simulink model "YMBOX_Control_Core"  (R2024b)
settings: Solver=FixedStepDiscrete  StartTime=0.0  StopTime=3  RelTol=1e-3
PreLoadFcn:
  | run(fullfile(fileparts(get_param(bdroot,'FileName')), 'YMBOX_Deluxe_init.m'));
InitFcn:
  | YMBOX_InitializeModel('core',bdroot);
model workspace (MAT data in the model file):
  KuMDAS_ObserverBuildVariant : Simulink.Parameter (value not decoded)
undefined symbols (not defined in the file or in its folder): CeMDSM_DrvModeIfStart_enum, CeMDSM_DrvModeSpdSens_enum, CeMDSM_DrvModeSpdSmo_enum, CeMDSM_DrvModeTrq_enum, Cf_CONTROL_TASK_TIME_S, KbMDAS_SmoDeadTimeCompEnable_flg, KbMDSA_ActiveInverterCompEnable_flg, KbMDSA_UnifiedVoltageLimitEnable_flg, KbMDSP_DCBusVoltReportFilterEnable_flg, KbMDTM_DAxisPriorityInFW_flg, KbMDTM_FieldWeakeningEnable_flg, KbMDTM_FinalIqAntiWindupEnable_flg, KbMDTM_SensorlessFieldWeakeningEnable_flg, KbMDTM_TorquePriorityBelowBase_flg, KbMDTM_UnifiedConstraintEnable_flg, KfMDAS_ControlCountToElecRad_NULL, KfMDAS_IfAccel_rpms, KfMDAS_IfAlignTime_s, KfMDAS_IfBlendTime_s, KfMDAS_IfSwitchSpd_rpm, KfMDAS_NativeCountToMechRad_NULL, KfMDAS_ObserverExitRatio_NULL, KfMDAS_SlsCtrlPeriod_s, KfMDAS_SlsEAngleInit_rad, KfMDAS_SlsElecSpdMax_rads, KfMDAS_SlsElecSpdMin_rads, KfMDAS_SlsTwoPi_rad, KfMDAS_SmoAngleOffset_rad, KfMDAS_SmoCurrentZohCoefA_NULL, KfMDAS_SmoCurrentZohCoefB_AperV, KfMDAS_SmoDeadTimeCurrentBoundary_A, KfMDAS_SmoDeadTimeDuty_NULL, KfMDAS_SmoDeadTimePolarity_NULL, KfMDAS_SmoDeviceDrop_V, KfMDAS_SmoEmfLpfCoefA_NULL, KfMDAS_SmoEmfLpfCoefB_NULL, KfMDAS_SmoEmfLpfInvPole_s, KfMDAS_SmoErrBoundaryMax_A, KfMDAS_SmoErrBoundarySpan_A, KfMDAS_SmoGainSchedAlpha_NULL, KfMDAS_SmoGainSchedAngleComp_rad, KfMDAS_SmoGainSchedEmfLow_V, KfMDAS_SmoGainSchedInvSpan_PerV, KfMDAS_SmoLdMinusLq_H, KfMDAS_SmoPllKiTs_NULL, KfMDAS_SmoPllKp_NULL, KfMDAS_SmoPllMinEmf_V, KfMDAS_SmoPllSpeedLpfAlpha_NULL, KfMDAS_SmoSlideGainMin_V, KfMDAS_SmoSlideGainSpan_V, KfMDAS_SmoSwitchSpd_rpm, KfMDAS_SmoTotalDelay_s, KfMDCC_DqSoftwareOverCurrentThreshold_A, KfMDCC_PiKcTsId_NULL, KfMDCC_PiKcTsIq_NULL, KfMDCC_PiKiTsId_NULL, KfMDCC_PiKiTsIq_NULL, KfMDCC_PiKpValueId_NULL, KfMDCC_PiKpValueIq_NULL, KfMDCC_PwmFreq_Hz ... (+84)
libraries: YMBOX_SharedMath_Lib x11, spsabctoAlphaBetaZeroLib x1
(part 3 of 8)

== system YMBOX_Control_Core/MDSP/Phase_Current_Conditioning ==
  phaseU_A : Inport  OutDataTypeStr=single
  phaseV_A : Inport  Port=2  OutDataTypeStr=single
  phaseW_A : Inport  Port=3  OutDataTypeStr=single
  phaseUError_flg : Inport  Port=4  OutDataTypeStr=boolean
  phaseVError_flg : Inport  Port=5  OutDataTypeStr=boolean
  phaseWError_flg : Inport  Port=6  OutDataTypeStr=boolean
  Invalid : Logic  Operator=OR  Inputs=3  IconShape=distinctive
  Pair0 : Logic  IconShape=distinctive
  Pair1 : Logic  IconShape=distinctive
  Pair2 : Logic  IconShape=distinctive
  Reconstruct0 : Sum  Inputs=--
  Reconstruct1 : Sum  Inputs=--
  Reconstruct2 : Sum  Inputs=--
  Safe0 : Switch  Criteria=u2 ~= 0
  Safe1 : Switch  Criteria=u2 ~= 0
  Safe2 : Switch  Criteria=u2 ~= 0
  Single0 : Switch  Criteria=u2 ~= 0
  Single1 : Switch  Criteria=u2 ~= 0
  Single2 : Switch  Criteria=u2 ~= 0
  Zero : Constant  Value=single(0)  OutDataTypeStr=single
  VfMDSP_PhaseUCurrentCtrl_A : Outport
  VfMDSP_PhaseVCurrentCtrl_A : Outport  Port=2
  VfMDSP_PhaseWCurrentCtrl_A : Outport  Port=3
  wires:
  phaseUError_flg/1 -> Single0/2, Pair0/1, Pair1/1
  Reconstruct0/1 -> Single0/1
  phaseU_A/1 -> Reconstruct2/1, Single0/3, Reconstruct1/1
  phaseVError_flg/1 -> Pair0/2, Pair2/1, Single1/2
  phaseWError_flg/1 -> Pair1/2, Pair2/2, Single2/2
  phaseV_A/1 -> Reconstruct2/2, Single1/3, Reconstruct0/1
  Pair0/1 -> Invalid/1
  phaseW_A/1 -> Single2/3, Reconstruct0/2, Reconstruct1/2
  Pair1/1 -> Invalid/2
  Pair2/1 -> Invalid/3
  Reconstruct2/1 -> Single2/1
  Reconstruct1/1 -> Single1/1
  Single0/1 -> Safe0/3
  Zero/1 -> Safe0/1, Safe2/1, Safe1/1
  Invalid/1 -> Safe0/2, Safe2/2, Safe1/2
  Single2/1 -> Safe2/3
  Single1/1 -> Safe1/3
  Safe0/1 -> VfMDSP_PhaseUCurrentCtrl_A/1
  Safe2/1 -> VfMDSP_PhaseWCurrentCtrl_A/1
  Safe1/1 -> VfMDSP_PhaseVCurrentCtrl_A/1

== system YMBOX_Control_Core/MDSP/Resolver_Processing ==
  VuMINP_ResolverPositionRaw_NULL : Inport  OutDataTypeStr=uint32
  ControlAngleCounts : Constant  Value=KfPLL_ControlAngleCounts_NULL
  ElectricAngle_ToUint16 : DataTypeConversion  OutDataTypeStr=uint16
  MechanicalRaw_Uint32 : SignalConversion  OverrideOpt=off
  NativeToElectricalCounts : Gain  Gain=KfPLL_PolePairsNativeToControl_NULL  OutDataTypeStr=single  SaturateOnIntegerOverflow=on
  Resolver_Output_Bus : BusCreator  Inputs=2  OutDataTypeStr=Bus: Resolver_Output  NonVirtualBus=on
      settings: InheritFromInputs=off
  WrapElectricalCount : Math  Operator=mod  OutDataTypeStr=uint16
  Resolver_Output : Outport  OutDataTypeStr=Bus: Resolver_Output
  wires:
  Resolver_Output_Bus/1 -> Resolver_Output/1  "Resolver_Output"
  MechanicalRaw_Uint32/1 -> Resolver_Output_Bus/2  "VuMDSP_MotMechAngleRaw_NULL"
  ElectricAngle_ToUint16/1 -> Resolver_Output_Bus/1  "VuMDSP_MotEAngle_NULL"
  VuMINP_ResolverPositionRaw_NULL/1 -> NativeToElectricalCounts/1, MechanicalRaw_Uint32/1
  NativeToElectricalCounts/1 -> WrapElectricalCount/1
  ControlAngleCounts/1 -> WrapElectricalCount/2
  WrapElectricalCount/1 -> ElectricAngle_ToUint16/1

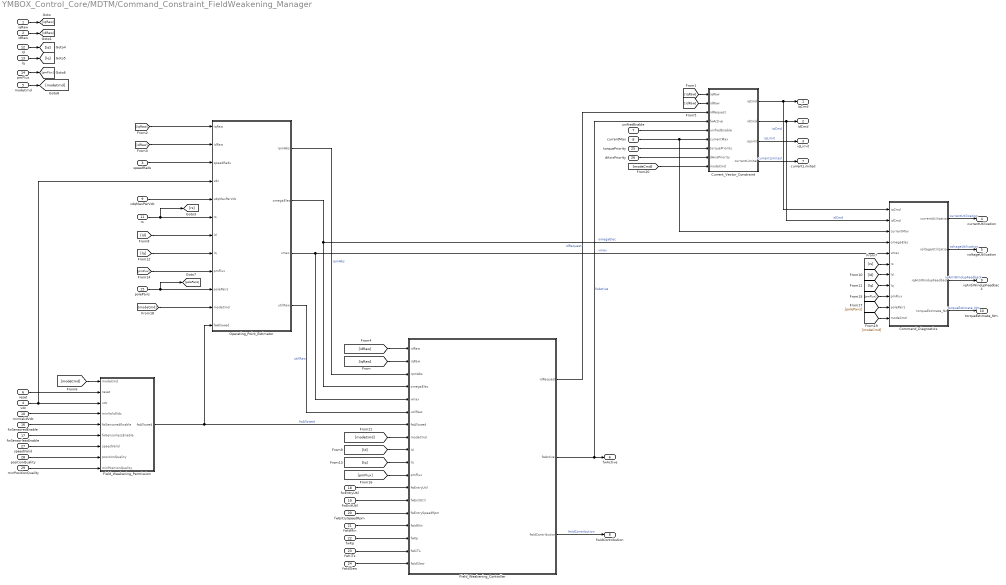
== system YMBOX_Control_Core/MDTM/Command_Constraint_FieldWeakening_Manager ==
  iqRaw : Inport
  idRaw : Inport  Port=2
  speedRads : Inport  Port=3
  vdc : Inport  Port=4
  modeCmd : Inport  Port=5
  reset : Inport  Port=6
  unifiedEnable : Inport  Port=7
  currentMax : Inport  Port=8
  vdqMaxPerVdc : Inport  Port=9
  minValidVdc : Inport  Port=10
  rs : Inport  Port=11
  ld : Inport  Port=12
  lq : Inport  Port=13
  pmFlux : Inport  Port=14
  polePairs : Inport  Port=15
  fwSensoredEnable : Inport  Port=16
  fwSensorlessEnable : Inport  Port=17
  fwEntryUtil : Inport  Port=18
  fwExitUtil : Inport  Port=19
  fwEntrySpeedRpm : Inport  Port=20
  fwIdMin : Inport  Port=21
  fwKp : Inport  Port=22
  fwKiTs : Inport  Port=23
  fwIdSlew : Inport  Port=24
  torquePriority : Inport  Port=25
  dAxisPriority : Inport  Port=26
  speedValid : Inport  Port=27
  positionQuality : Inport  Port=28
  minPositionQuality : Inport  Port=29
  Command_Diagnostics : Subsystem
  Current_Vector_Constraint : Subsystem
  Field_Weakening_Controller : Subsystem
  Field_Weakening_Permission : Subsystem
  Operating_Point_Estimator : Subsystem
  iqCmd : Outport
  idCmd : Outport  Port=2
  iqLimit : Outport  Port=3
  currentUtilization : Outport  Port=4
  voltageUtilization : Outport  Port=5
  fwActive : Outport  Port=6
  currentLimited : Outport  Port=7
  fwIdContribution : Outport  Port=8
  iqAntiWindupFeedback : Outport  Port=9
  torqueEstimate_Nm : Outport  Port=10
  wires:
  vdqMaxPerVdc/1 -> Operating_Point_Estimator/5(vdqMaxPerVdc)
  reset/1 -> Field_Weakening_Permission/2(reset)
  Operating_Point_Estimator/2(omegaElec) -> Field_Weakening_Controller/4(omegaElec), Command_Diagnostics/4(omegaElec)  "omegaElec"
  Command_Diagnostics/2(voltageUtilization) -> voltageUtilization/1  "voltageUtilization"
  vdc/1 -> Operating_Point_Estimator/4(vdc), Field_Weakening_Permission/3(vdc)
  speedRads/1 -> Operating_Point_Estimator/3(speedRads)
  Command_Diagnostics/4(torqueEstimate_Nm) -> torqueEstimate_Nm/1  "torqueEstimate_Nm"
  Operating_Point_Estimator/4(utilRaw) -> Field_Weakening_Controller/6(utilRaw)  "utilRaw"
  rs/1 -> [rs], Operating_Point_Estimator/6(rs)
  Current_Vector_Constraint/4(currentLimited) -> currentLimited/1  "currentLimited"
  Field_Weakening_Controller/2(fwActive) -> fwActive/1, Current_Vector_Constraint/4(fwActive)  "fwActive"
  polePairs/1 -> [polePairs], Operating_Point_Estimator/10(polePairs)
  Operating_Point_Estimator/1(rpmAbs) -> Field_Weakening_Controller/3(rpmAbs)  "rpmAbs"
  Operating_Point_Estimator/3(vmax) -> Field_Weakening_Controller/5(vmax), Command_Diagnostics/5(vmax)  "vmax"
  fwEntryUtil/1 -> Field_Weakening_Controller/12(fwEntryUtil)
  Current_Vector_Constraint/2(idCmd) -> Command_Diagnostics/2(idCmd), idCmd/1  "idCmd"
  fwExitUtil/1 -> Field_Weakening_Controller/13(fwExitUtil)
  fwEntrySpeedRpm/1 -> Field_Weakening_Controller/14(fwEntrySpeedRpm)
  fwIdMin/1 -> Field_Weakening_Controller/15(fwIdMin)
  fwKp/1 -> Field_Weakening_Controller/16(fwKp)
  fwKiTs/1 -> Field_Weakening_Controller/17(fwKiTs)
  fwIdSlew/1 -> Field_Weakening_Controller/18(fwIdSlew)
  unifiedEnable/1 -> Current_Vector_Constraint/5(unifiedEnable)
  torquePriority/1 -> Current_Vector_Constraint/7(torquePriority)
  dAxisPriority/1 -> Current_Vector_Constraint/8(dAxisPriority)
  currentMax/1 -> Command_Diagnostics/3(currentMax), Current_Vector_Constraint/6(currentMax)
  Field_Weakening_Controller/1(idRequest) -> Current_Vector_Constraint/3(idRequest)  "idRequest"
  Command_Diagnostics/1(currentUtilization) -> currentUtilization/1  "currentUtilization"
  Field_Weakening_Controller/3(fwIdContribution) -> fwIdContribution/1  "fwIdContribution"
  Current_Vector_Constraint/1(iqCmd) -> Command_Diagnostics/1(iqCmd), iqCmd/1  "iqCmd"
  Current_Vector_Constraint/3(iqLimit) -> iqLimit/1  "iqLimit"
  Command_Diagnostics/3(iqAntiWindupFeedback) -> iqAntiWindupFeedback/1  "iqAntiWindupFeedback"
  iqRaw/1 -> [iqRaw]
  [iqRaw] -> Field_Weakening_Controller/2(iqRaw)
  [iqRaw] -> Current_Vector_Constraint/1(iqRaw)
  [iqRaw] -> Operating_Point_Estimator/1(iqRaw)
  idRaw/1 -> [idRaw]
  [idRaw] -> Operating_Point_Estimator/2(idRaw)
  [idRaw] -> Field_Weakening_Controller/1(idRaw)
  [idRaw] -> Current_Vector_Constraint/2(idRaw)
  [rs] -> Command_Diagnostics/6(rs)
  ld/1 -> [ld]
  [ld] -> Operating_Point_Estimator/7(ld)
  [ld] -> Field_Weakening_Controller/9(ld)
  [ld] -> Command_Diagnostics/7(ld)
  lq/1 -> [lq]
  [lq] -> Command_Diagnostics/8(lq)
  [lq] -> Operating_Point_Estimator/8(lq)
  [lq] -> Field_Weakening_Controller/10(lq)
  pmFlux/1 -> [pmFlux]
  [pmFlux] -> Operating_Point_Estimator/9(pmFlux)
  [pmFlux] -> Command_Diagnostics/9(pmFlux)
  [pmFlux] -> Field_Weakening_Controller/11(pmFlux)
  [polePairs] -> Command_Diagnostics/10(polePairs)
  modeCmd/1 -> [modeCmd]
  [modeCmd] -> Operating_Point_Estimator/11(modeCmd)
  [modeCmd] -> Command_Diagnostics/11(modeCmd)
  [modeCmd] -> Current_Vector_Constraint/9(modeCmd)
  [modeCmd] -> Field_Weakening_Controller/8(modeCmd)
  minValidVdc/1 -> Field_Weakening_Permission/4(minValidVdc)
  fwSensoredEnable/1 -> Field_Weakening_Permission/5(fwSensoredEnable)
  fwSensorlessEnable/1 -> Field_Weakening_Permission/6(fwSensorlessEnable)
  speedValid/1 -> Field_Weakening_Permission/7(speedValid)
  positionQuality/1 -> Field_Weakening_Permission/8(positionQuality)
  minPositionQuality/1 -> Field_Weakening_Permission/9(minPositionQuality)
  Field_Weakening_Permission/1(fwAllowed) -> Operating_Point_Estimator/12(fwAllowed), Field_Weakening_Controller/7(fwAllowed)  "fwAllowed"
  [modeCmd] -> Field_Weakening_Permission/1(modeCmd)

== system YMBOX_Control_Core/MDTM/MDTM ==
  note: 1) Add Subsystem or Model blocks as valid variant choices.
      | 2) You cannot connect blocks at this level. At simulation, connectivity is automatically
      | determined, based on the active variant and port name matching.
  VeMDTM_DrvModeCmd_enum : Inport
  VeMDTM_DrvModeReq_enum : Inport  Port=2
  VfMDTM_SpdCmd_rpm : Inport  Port=3
  VfMDTM_TrqCmd_Nm : Inport  Port=4
  VbMDCC_PiReset_flg : Inport  Port=5
  VfMDCC_TestUalphaUdId_NULL : Inport  Port=6
  VfMDTM_TestUbetaUqIq_NULL : Inport  Port=7
  VfMDTM_HandoverBlend_NULL : Inport  Port=8
  VfMDTM_HandoverElecAngleDelta_rad : Inport  Port=9
  VfMDTM_MotMechSpdFiltered_rads : Inport  Port=10
  VfMDTM_MotElecAngle_rad : Inport  Port=11
  VfMDTM_PhaseUCur_A : Inport  Port=12
  VfMDTM_PhaseVCur_A : Inport  Port=13
  VfMDTM_PhaseWCur_A : Inport  Port=14
  VfMDTM_ExecutionScale_NULL : Inport  Port=15  OutDataTypeStr=single
  MDTM_SMO : Subsystem  TreatAsAtomicUnit=on  VariantControl=KuMDAS_ObserverBuildVariant == 1
      settings: AttributesFormatString=PRODUCT TORQUE/SPEED CONTROL\nMODE 6: SENSORLESS SPEED
  MDTM_SensoredOnly : Subsystem  TreatAsAtomicUnit=on  VariantControl=KuMDAS_ObserverBuildVariant == 0
      settings: AttributesFormatString=|
      | SENSORED ONLY
      | Original direct voltage/speed/torque modes 3/4/5
  MDTM_outputs : Outport

== system YMBOX_Control_Core/MDTM/MotorCurrentReferenceGenerator ==
  note: 1) Add Subsystem or Model blocks as valid variant choices.
      | 2) You cannot connect blocks at this level. At simulation, connectivity is automatically
      | determined, based on the active variant and port name matching.
  modeCmd_enum : Inport
  iqLegacy_A : Inport  Port=2
  idLegacy_A : Inport  Port=3
  handoverBlend_NULL : Inport  Port=4  OutDataTypeStr=single
  MotorCurrentReference_IPMSM : Subsystem  VariantControl=KuMDTM_MotorCurrentReferenceVariant == 1
  MotorCurrentReference_SPMSM : Subsystem  VariantControl=KuMDTM_MotorCurrentReferenceVariant == 0
  iqReference_A : Outport
  idReference_A : Outport  Port=2
  torqueRequest_Nm : Outport  Port=3
  mtpaActive_flg : Outport  Port=4

== system YMBOX_Control_Core/MDAS/IF_Startup_Internal/IF_Startup_SMO ==
  VeMDAS_DrvModeCmd_enum : Inport
  VeMDAS_DrvModeReq_enum : Inport  Port=2
  VfMDAS_TargetSpd_rpm : Inport  Port=3
  VfMDAS_SmoElecSpd_rads : Inport  Port=4
  VfMDAS_SmoElecAngle_rad : Inport  Port=5
  VfMDAS_SmoEmfMag_V : Inport  Port=6
  VfMDAS_SmoPllPhaseErr_NULL : Inport  Port=7
  SMO_ProductMode_Core : Stateflow chart  TreatAsAtomicUnit=on
  VfMDAS_IfMechSpd_rads : Outport
  VfMDAS_IfMechSpdAbs_rads : Outport  Port=2
  VfMDAS_IfElecAngle_rad : Outport  Port=3
  VfMDAS_SmoMechSpd_rads : Outport  Port=4
  VfMDAS_SmoMechSpdAbs_rads : Outport  Port=5
  VbMDAS_SmoReady_flg : Outport  Port=6
  VfMDAS_SmoAlignedElecAngle_rad : Outport  Port=7
  VfMDAS_HandoverBlend_NULL : Outport  Port=8
  VfMDAS_HandoverElecAngleDelta_rad : Outport  Port=9
  wires:
  VeMDAS_DrvModeCmd_enum/1 -> SMO_ProductMode_Core/1(VeMDAS_DrvModeCmd_enum)
  VeMDAS_DrvModeReq_enum/1 -> SMO_ProductMode_Core/2(VeMDAS_DrvModeReq_enum)
  SMO_ProductMode_Core/2(VfMDAS_IfMechSpdAbs_rads) -> VfMDAS_IfMechSpdAbs_rads/1
  SMO_ProductMode_Core/1(VfMDAS_IfMechSpd_rads) -> VfMDAS_IfMechSpd_rads/1
  VfMDAS_TargetSpd_rpm/1 -> SMO_ProductMode_Core/3(VfMDAS_TargetSpd_rpm)
  VfMDAS_SmoElecSpd_rads/1 -> SMO_ProductMode_Core/4(VfMDAS_SmoElecSpd_rads)
  VfMDAS_SmoElecAngle_rad/1 -> SMO_ProductMode_Core/5(VfMDAS_SmoElecAngle_rad)
  VfMDAS_SmoEmfMag_V/1 -> SMO_ProductMode_Core/6(VfMDAS_SmoEmfMag_V)
  VfMDAS_SmoPllPhaseErr_NULL/1 -> SMO_ProductMode_Core/7(VfMDAS_SmoPllPhaseErr_NULL)
  SMO_ProductMode_Core/6(VbMDAS_SmoReady_flg) -> VbMDAS_SmoReady_flg/1
  SMO_ProductMode_Core/5(VfMDAS_SmoMechSpdAbs_rads) -> VfMDAS_SmoMechSpdAbs_rads/1
  SMO_ProductMode_Core/4(VfMDAS_SmoMechSpd_rads) -> VfMDAS_SmoMechSpd_rads/1
  SMO_ProductMode_Core/3(VfMDAS_IfElecAngle_rad) -> VfMDAS_IfElecAngle_rad/1
  SMO_ProductMode_Core/9(VfMDAS_HandoverElecAngleDelta_rad) -> VfMDAS_HandoverElecAngleDelta_rad/1
  SMO_ProductMode_Core/8(VfMDAS_HandoverBlend_NULL) -> VfMDAS_HandoverBlend_NULL/1
  SMO_ProductMode_Core/7(VfMDAS_SmoAlignedElecAngle_rad) -> VfMDAS_SmoAlignedElecAngle_rad/1

== system YMBOX_Control_Core/MDAS/IF_Startup_Internal/IF_Startup_SensoredOnly ==
  VeMDAS_DrvModeCmd_enum : Inport
  VeMDAS_DrvModeReq_enum : Inport  Port=2
  VfMDAS_TargetSpd_rpm : Inport  Port=3
  VfMDAS_SmoElecSpd_rads : Inport  Port=4
  VfMDAS_SmoElecAngle_rad : Inport  Port=5
  VfMDAS_SmoEmfMag_V : Inport  Port=6
  VfMDAS_SmoPllPhaseErr_NULL : Inport  Port=7
  FalseBoolean : Constant  Value=false  OutDataTypeStr=boolean
  TerminateInput01 : Terminator
  TerminateInput02 : Terminator
  TerminateInput03 : Terminator
  TerminateInput06 : Terminator
  TerminateInput07 : Terminator
  TerminateInput08 : Terminator
  TerminateInput09 : Terminator
  ZeroSingle : Constant  Value=single(0)  OutDataTypeStr=single
  VfMDAS_IfMechSpd_rads : Outport
  VfMDAS_IfMechSpdAbs_rads : Outport  Port=2
  VfMDAS_IfElecAngle_rad : Outport  Port=3
  VfMDAS_SmoMechSpd_rads : Outport  Port=4
  VfMDAS_SmoMechSpdAbs_rads : Outport  Port=5
  VbMDAS_SmoReady_flg : Outport  Port=6
  VfMDAS_SmoAlignedElecAngle_rad : Outport  Port=7
  VfMDAS_HandoverBlend_NULL : Outport  Port=8
  VfMDAS_HandoverElecAngleDelta_rad : Outport  Port=9
  wires:
  VfMDAS_TargetSpd_rpm/1 -> TerminateInput03/1
  VfMDAS_SmoPllPhaseErr_NULL/1 -> TerminateInput09/1
  VfMDAS_SmoElecAngle_rad/1 -> TerminateInput07/1
  VfMDAS_SmoEmfMag_V/1 -> TerminateInput08/1
  VeMDAS_DrvModeReq_enum/1 -> TerminateInput02/1
  VfMDAS_SmoElecSpd_rads/1 -> TerminateInput06/1
  VeMDAS_DrvModeCmd_enum/1 -> TerminateInput01/1
  ZeroSingle/1 -> VfMDAS_SmoMechSpd_rads/1, VfMDAS_HandoverElecAngleDelta_rad/1, VfMDAS_HandoverBlend_NULL/1, VfMDAS_IfElecAngle_rad/1, VfMDAS_SmoMechSpdAbs_rads/1, VfMDAS_IfMechSpdAbs_rads/1, VfMDAS_IfMechSpd_rads/1, VfMDAS_SmoAlignedElecAngle_rad/1
  FalseBoolean/1 -> VbMDAS_SmoReady_flg/1

== system YMBOX_Control_Core/MDAS/MDAS_DriveModeRoute_Variant/MDAS_Route_SMO ==
  <VeMDSM_DrvModeCmd_enum> : Inport
  <VuMDSP_MotMechAngleRaw_NULL> : Inport  Port=2
  VfMDAS_IfMechSpdAbs_rads : Inport  Port=3
  VfMDAS_IfMechSpd_rads : Inport  Port=4
  VfMDAS_SmoMechSpdAbs_rads : Inport  Port=5
  VfMDAS_SmoMechSpd_rads : Inport  Port=6
  VfMDAS_IfElecAngle_rad : Inport  Port=7
  VfMDAS_SmoAlignedElecAngle_rad : Inport  Port=8
  Action_DefaultZero : Subsystem  TreatAsAtomicUnit=on
  Action_IF_Startup : Subsystem  TreatAsAtomicUnit=on
  Action_SMO_ClosedLoop : Subsystem  TreatAsAtomicUnit=on
      settings: AttributesFormatString=INTERNAL 17: SMO CLOSED LOOP
  Merge : Merge  Inputs=4
  Merge3 : Merge  Inputs=4
  Selected_ElecAngle_Rad_Merge : Merge  Inputs=4
  Switch Case Action Subsystem : Subsystem  TreatAsAtomicUnit=on
  Switch_Case_InternalMode : SwitchCase  CaseConditions={[CeMDSM_DrvModeVoltAB_enum,CeMDSM_DrvModeVoltDQ_enum,CeMDSM_DrvModeCurrDQ_enum,CeMDSM_DrvModeSpdSens_enum,CeMDSM_DrvModeTrq_enum],CeMDSM_DrvModeIfStart_enum,CeMDSM_DrvModeSpdSmo_enum}
  VfMDAS_MotMechSpdFiltered_rads : Outport
  VfMDAS_MotMechSpdFilteredAbs_rads : Outport  Port=2
  VfMDAS_SelectedElecAngle_rad : Outport  Port=3
  wires:
  Switch_Case_InternalMode/4 -> Action_DefaultZero/Action
  <VeMDSM_DrvModeCmd_enum>/1 -> Switch_Case_InternalMode/1
  VfMDAS_IfElecAngle_rad/1 -> Action_IF_Startup/3(VfMDAS_SourceElecAngle_rad)
  Switch_Case_InternalMode/2 -> Action_IF_Startup/Action
  Switch_Case_InternalMode/3 -> Action_SMO_ClosedLoop/Action
  Action_IF_Startup/3(VfMDAS_SelectedElecAngle_rad) -> Selected_ElecAngle_Rad_Merge/2
  <VuMDSP_MotMechAngleRaw_NULL>/1 -> Switch Case Action Subsystem/1(VuMDSP_MotMechAngleRaw_NULL)
  VfMDAS_IfMechSpdAbs_rads/1 -> Action_IF_Startup/2(VfMDAS_SourceMechSpdAbs_rads)
  VfMDAS_SmoMechSpdAbs_rads/1 -> Action_SMO_ClosedLoop/2(VfMDAS_SourceMechSpdAbs_rads)
  VfMDAS_IfMechSpd_rads/1 -> Action_IF_Startup/1(VfMDAS_SourceMechSpd_rads)
  Switch_Case_InternalMode/1 -> Switch Case Action Subsystem/Action
  VfMDAS_SmoMechSpd_rads/1 -> Action_SMO_ClosedLoop/1(VfMDAS_SourceMechSpd_rads)
  Action_SMO_ClosedLoop/3(VfMDAS_SelectedElecAngle_rad) -> Selected_ElecAngle_Rad_Merge/3
  Action_SMO_ClosedLoop/2(VfMDAS_MotMechSpdFilteredAbs_rads) -> Merge3/3
  Action_SMO_ClosedLoop/1(VfMDAS_MotMechSpdFiltered_rads) -> Merge/3
  VfMDAS_SmoAlignedElecAngle_rad/1 -> Action_SMO_ClosedLoop/3(VfMDAS_SourceElecAngle_rad)
  Switch Case Action Subsystem/3(VfMDAS_SelectedElecAngle_rad) -> Selected_ElecAngle_Rad_Merge/1
  Switch Case Action Subsystem/2(VfMDAS_MotMechSpdFilteredAbs_rads) -> Merge3/1
  Switch Case Action Subsystem/1(VfMDAS_MotMechSpdFiltered_rads) -> Merge/1
  Action_IF_Startup/2(VfMDAS_MotMechSpdFilteredAbs_rads) -> Merge3/2
  Action_IF_Startup/1(VfMDAS_MotMechSpdFiltered_rads) -> Merge/2
  Action_DefaultZero/2(VfMDAS_MotMechSpdFilteredAbs_rads) -> Merge3/4
  Action_DefaultZero/1(VfMDAS_MotMechSpdFiltered_rads) -> Merge/4
  Action_DefaultZero/3(VfMDAS_SelectedElecAngle_rad) -> Selected_ElecAngle_Rad_Merge/4
  Merge/1 -> VfMDAS_MotMechSpdFiltered_rads/1  "VfMDAS_MotMechSpdFiltered_rads"
  Merge3/1 -> VfMDAS_MotMechSpdFilteredAbs_rads/1  "VfMDAS_MotMechSpdFilteredAbs_rads"
  Selected_ElecAngle_Rad_Merge/1 -> VfMDAS_SelectedElecAngle_rad/1  "VfMDAS_SelectedElecAngle_rad"

== system YMBOX_Control_Core/MDAS/MDAS_DriveModeRoute_Variant/MDAS_Route_SensoredOnly ==
  <VeMDSM_DrvModeCmd_enum> : Inport
  <VuMDSP_MotMechAngleRaw_NULL> : Inport  Port=2
  VfMDAS_IfMechSpdAbs_rads : Inport  Port=3
  VfMDAS_IfMechSpd_rads : Inport  Port=4
  VfMDAS_SmoMechSpdAbs_rads : Inport  Port=5
  VfMDAS_SmoMechSpd_rads : Inport  Port=6
  VfMDAS_IfElecAngle_rad : Inport  Port=7
  VfMDAS_SmoAlignedElecAngle_rad : Inport  Port=8
  Enabled : DataTypeConversion  OutDataTypeStr=boolean
  Sensored_AngleSpeed : Subsystem  TreatAsAtomicUnit=on
  TerminateInput05 : Terminator
  TerminateInput06 : Terminator
  TerminateInput08 : Terminator
  TerminateInput09 : Terminator
  TerminateInput11 : Terminator
  TerminateInput12 : Terminator
  VfMDAS_MotMechSpdFiltered_rads : Outport
  VfMDAS_MotMechSpdFilteredAbs_rads : Outport  Port=2
  VfMDAS_SelectedElecAngle_rad : Outport  Port=3
  wires:
  VfMDAS_SmoMechSpdAbs_rads/1 -> TerminateInput08/1
  Sensored_AngleSpeed/1(VfMDAS_MotMechSpdFiltered_rads) -> VfMDAS_MotMechSpdFiltered_rads/1
  VfMDAS_SmoAlignedElecAngle_rad/1 -> TerminateInput12/1
  VfMDAS_IfMechSpdAbs_rads/1 -> TerminateInput05/1
  <VuMDSP_MotMechAngleRaw_NULL>/1 -> Sensored_AngleSpeed/1(VuMDSP_MotMechAngleRaw_NULL)
  VfMDAS_SmoMechSpd_rads/1 -> TerminateInput09/1
  VfMDAS_IfElecAngle_rad/1 -> TerminateInput11/1
  VfMDAS_IfMechSpd_rads/1 -> TerminateInput06/1
  Sensored_AngleSpeed/3(VfMDAS_SelectedElecAngle_rad) -> VfMDAS_SelectedElecAngle_rad/1
  Sensored_AngleSpeed/2(VfMDAS_MotMechSpdFilteredAbs_rads) -> VfMDAS_MotMechSpdFilteredAbs_rads/1
  <VeMDSM_DrvModeCmd_enum>/1 -> Enabled/1
  Enabled/1 -> Sensored_AngleSpeed/Reset

== system YMBOX_Control_Core/MDAS/Sensorless_FluxMRAS/Observer_Variant0_SensoredOnly ==
  MDSP_outputs : Inport
  MDSA_outputs : Inport  Port=2
  MDSM_outputs : Inport  Port=3
  Terminate_MDSA_outputs : Terminator
  Terminate_MDSP_outputs : Terminator
  UnusedMode : Terminator
  ZeroSingle : Constant  Value=single(0)  OutDataTypeStr=single
  VfMDAS_SmoElecAngle_rad : Outport
  VfMDAS_SmoElecSpd_rads : Outport  Port=2
  VfMDAS_SmoEmfMag_V : Outport  Port=3
  VfMDAS_SmoPllPhaseErr_NULL : Outport  Port=4
  wires:
  MDSP_outputs/1 -> Terminate_MDSP_outputs/1
  MDSA_outputs/1 -> Terminate_MDSA_outputs/1
  ZeroSingle/1 -> VfMDAS_SmoPllPhaseErr_NULL/1, VfMDAS_SmoEmfMag_V/1, VfMDAS_SmoElecSpd_rads/1, VfMDAS_SmoElecAngle_rad/1
  MDSM_outputs/1 -> UnusedMode/1

== system YMBOX_Control_Core/MDAS/Sensorless_FluxMRAS/Observer_Variant1_SMO ==
  MDSP_outputs : Inport
  MDSA_outputs : Inport  Port=2
  MDSM_outputs : Inport  Port=3
  Cast_SMO_AngleRad_single : DataTypeConversion  OutDataTypeStr=single  SaturateOnIntegerOverflow=off  RndMeth=Floor
  Cast_SMO_ElecSpeed_single : DataTypeConversion  OutDataTypeStr=single  SaturateOnIntegerOverflow=off  RndMeth=Floor
  Cast_SMO_EmfMag_single : DataTypeConversion  OutDataTypeStr=single  RndMeth=Round  SaturateOnIntegerOverflow=off
  Cast_SMO_PllPhaseErr_single : DataTypeConversion  OutDataTypeStr=single  RndMeth=Round  SaturateOnIntegerOverflow=off
  Cast_VoltageAlphaBetaZero : DataTypeConversion  OutDataTypeStr=single  SaturateOnIntegerOverflow=off  RndMeth=Floor
  Current_abc_to_AlphaBetaZero : spsabctoAlphaBetaZeroLib/abc to Alpha-Beta-Zero
  Mux_Iabc : Mux  Inputs=3
  Observer_RunState : Subsystem
  SMO_AdaptiveInjectionPhase : Gain  Gain=KfMDAS_SmoGainSchedAngleComp_rad
  SMO_AngleCompSum : Sum  Inputs=++++++
  SMO_AngleOffset : Constant  Value=single(KfMDAS_SmoAngleOffset_rad)  OutDataTypeStr=single
  SMO_AngleWrap : Math  Operator=mod
  SMO_DelayPhaseAdvance : Gain  Gain=KfMDAS_SmoTotalDelay_s
  SMO_EmfLpfInvPole : Constant  Value=KfMDAS_SmoEmfLpfInvPole_s
  SMO_LpfPhaseAdvance : YMBOX_SharedMath_Lib/Atan_Service  SystemSampleTime=-1  VariantActivationTime=update diagram  AllowFlexibleInterface=on  Latency=0  AutoFrameSizeCalculation=off
  SMO_Observer : Subsystem
  SMO_RotationDirectionOffset : Subsystem
  SMO_SpdByLpfPole : Product  Inputs=**
  SMO_TwoPi_Out : Constant  Value=single(KfMDAS_SlsTwoPi_rad)  OutDataTypeStr=single
  Select_PhaseCurrents : BusSelector  OutputSignals=VfMDSP_PhaseUCurrentCtrl_A,VfMDSP_PhaseVCurrentCtrl_A,VfMDSP_PhaseWCurrentCtrl_A,VfMDSP_DCBusVoltCtrl_V
  Select_PwmDuty : BusSelector  OutputSignals=VfMDSA_PwmDutyCyclePhaseU_NULL,VfMDSA_PwmDutyCyclePhaseV_NULL,VfMDSA_PwmDutyCyclePhaseW_NULL
  Term_SMO_EmfAlpha : Terminator
  Term_SMO_EmfBeta : Terminator
  Voltage_AlphaBeta_Reconstruction : Subsystem
  VfMDAS_SmoElecAngle_rad : Outport
  VfMDAS_SmoElecSpd_rads : Outport  Port=2
  VfMDAS_SmoEmfMag_V : Outport  Port=3
  VfMDAS_SmoPllPhaseErr_NULL : Outport  Port=4
  wires:
  MDSA_outputs/1 -> Select_PwmDuty/1
  MDSP_outputs/1 -> Select_PhaseCurrents/1
  SMO_Observer/2(VfMDAS_SmoEmfAlpha_V) -> Term_SMO_EmfAlpha/1  "VfMDOB_SmoEmfAlpha_V"
  SMO_Observer/1(VfMDAS_SmoRawEAngle_rad) -> SMO_AngleCompSum/2  "VfMDOB_SmoElecAngle_rad"
  Select_PhaseCurrents/3 -> Mux_Iabc/3, Voltage_AlphaBeta_Reconstruction/6(PhaseCurrentW_A)  "<VfMDSP_PhaseWCurrentCtrl_A>"
  Current_abc_to_AlphaBetaZero/1 -> SMO_Observer/2(VfMDAS_SmoCurAlphaBetaZero_A)
  Select_PwmDuty/1 -> Voltage_AlphaBeta_Reconstruction/1(VfMDAS_SlsPwmDutyPhaseU_NULL)  "<VfMDSA_PwmDutyCyclePhaseU_NULL>"
  Select_PwmDuty/2 -> Voltage_AlphaBeta_Reconstruction/2(VfMDAS_SlsPwmDutyPhaseV_NULL)  "<VfMDSA_PwmDutyCyclePhaseV_NULL>"
  Select_PhaseCurrents/1 -> Mux_Iabc/1, Voltage_AlphaBeta_Reconstruction/4(PhaseCurrentU_A)  "<VfMDSP_PhaseUCurrentCtrl_A>"
  Select_PwmDuty/3 -> Voltage_AlphaBeta_Reconstruction/3(VfMDAS_SlsPwmDutyPhaseW_NULL)  "<VfMDSA_PwmDutyCyclePhaseW_NULL>"
  Select_PhaseCurrents/2 -> Mux_Iabc/2, Voltage_AlphaBeta_Reconstruction/5(PhaseCurrentV_A)  "<VfMDSP_PhaseVCurrentCtrl_A>"
  Select_PhaseCurrents/4 -> Voltage_AlphaBeta_Reconstruction/7(DcBusVoltage_V)  "<VfMDSP_DCBusVoltCtrl_V>"
  Voltage_AlphaBeta_Reconstruction/1(VfMDAS_SlsVoltAlphaBetaZero_V) -> Cast_VoltageAlphaBetaZero/1  "VfMDOB_VoltAlphaBetaZero_V"
  Mux_Iabc/1 -> Current_abc_to_AlphaBetaZero/1
  Cast_VoltageAlphaBetaZero/1 -> SMO_Observer/1(VfMDAS_SmoVoltAlphaBetaZero_V)
  SMO_Observer/6(VfMDAS_SmoPllPhaseErr_NULL) -> Cast_SMO_PllPhaseErr_single/1
  SMO_Observer/5(VfMDAS_SmoEmfMag_V) -> Cast_SMO_EmfMag_single/1
  SMO_Observer/4(VfMDAS_SmoRawElecSpd_rads) -> SMO_RotationDirectionOffset/1(electricalSpeed), SMO_DelayPhaseAdvance/1, Cast_SMO_ElecSpeed_single/1, SMO_SpdByLpfPole/1  "VfMDOB_SmoElecSpd_rads"
  SMO_Observer/3(VfMDAS_SmoEmfBeta_V) -> Term_SMO_EmfBeta/1  "VfMDOB_SmoEmfBeta_V"
  SMO_Observer/7(VfMDAS_SmoGainSchedule_NULL) -> SMO_AdaptiveInjectionPhase/1  "VfMDAS_SmoGainSchedule_NULL"
  SMO_DelayPhaseAdvance/1 -> SMO_AngleCompSum/1
  SMO_EmfLpfInvPole/1 -> SMO_SpdByLpfPole/2
  Cast_SMO_ElecSpeed_single/1 -> VfMDAS_SmoElecSpd_rads/1  "VfMDAS_SmoElecSpd_rads"
  Cast_SMO_PllPhaseErr_single/1 -> VfMDAS_SmoPllPhaseErr_NULL/1
  Cast_SMO_EmfMag_single/1 -> VfMDAS_SmoEmfMag_V/1
  SMO_AngleOffset/1 -> SMO_AngleCompSum/3
  SMO_AdaptiveInjectionPhase/1 -> SMO_AngleCompSum/5  "VfMDAS_SmoAdaptivePhaseComp_rad"
  Cast_SMO_AngleRad_single/1 -> VfMDAS_SmoElecAngle_rad/1  "VfMDAS_SmoElecAngle_rad"
  SMO_SpdByLpfPole/1 -> SMO_LpfPhaseAdvance/1
  SMO_LpfPhaseAdvance/1 -> SMO_AngleCompSum/4
  MDSM_outputs/1 -> Observer_RunState/1(MDSM_outputs)
  Observer_RunState/1(Active) -> SMO_Observer/Reset
  SMO_RotationDirectionOffset/1(angleOffset) -> SMO_AngleCompSum/6
  SMO_AngleCompSum/1 -> SMO_AngleWrap/1
  SMO_TwoPi_Out/1 -> SMO_AngleWrap/2
  SMO_AngleWrap/1 -> Cast_SMO_AngleRad_single/1

== system YMBOX_Control_Core/MDCC/MDCC_Subsystem/Clarke ==
  note: Phase validity and reconstruction are owned by MDSP; Clarke consumes the shared control-current triplet.
  VfMDCC_UCur_A : Inport
  VfMDCC_VCur_A : Inport  Port=2
  VfMDCC_WCur_A : Inport  Port=3
  Difference : Sum  Inputs=+-
  Scale : Gain  Gain=single(0.57735)
  VfMDCC_AlphaCur_A : Outport
  VfMDCC_BetaCur_A : Outport  Port=2
  wires:
  VfMDCC_UCur_A/1 -> VfMDCC_AlphaCur_A/1
  VfMDCC_VCur_A/1 -> Difference/1
  VfMDCC_WCur_A/1 -> Difference/2
  Difference/1 -> Scale/1
  Scale/1 -> VfMDCC_BetaCur_A/1

== system YMBOX_Control_Core/MDCC/MDCC_Subsystem/DqSoftwareOverCurrent_Diagnostic ==
  VfMDCC_DCur_A : Inport
  VfMDCC_QCur_A : Inport  Port=2
  CountWhenDqCurrentExceeded : Subsystem  TreatAsAtomicUnit=on
  CountWhenDqCurrentNormal : Subsystem  TreatAsAtomicUnit=on
  Current_Magnitude_Squared : Subsystem
  DqSoftwareOverCurrentCountNext : Merge
  DqSoftwareOverCurrentCountState : Delay  DelayLength=1  InitialCondition=0
  DqSoftwareOverCurrentThresholdSq_A2 : Constant  Value=KfMDCC_DqSoftwareOverCurrentThreshold_A*KfMDCC_DqSoftwareOverCurrentThreshold_A
  If : If  NumInputs=2  IfExpression=u1 > u2 | u1 ~= u1
  VbMDCC_DqSoftwareOverCurrent_flg : Outport
  wires:
  DqSoftwareOverCurrentCountNext/1 -> DqSoftwareOverCurrentCountState/1
  CountWhenDqCurrentExceeded/2(VuMDCC_DqSoftwareOverCurrentCountNew_cnt) -> DqSoftwareOverCurrentCountNext/1
  If/2 -> CountWhenDqCurrentNormal/Action
  CountWhenDqCurrentNormal/1(VuMDCC_DqSoftwareOverCurrentCountNew_cnt) -> DqSoftwareOverCurrentCountNext/2
  DqSoftwareOverCurrentCountState/1 -> CountWhenDqCurrentExceeded/1(VuMDCC_DqSoftwareOverCurrentCount_cnt), CountWhenDqCurrentNormal/1(VuMDCC_DqSoftwareOverCurrentCount_cnt)
  If/1 -> CountWhenDqCurrentExceeded/Action
  CountWhenDqCurrentExceeded/1(VbMDCC_DqSoftwareOverCurrent_flg) -> VbMDCC_DqSoftwareOverCurrent_flg/1  "VbMDCC_DqSoftwareOverCurrent_flg"
  DqSoftwareOverCurrentThresholdSq_A2/1 -> If/2
  VfMDCC_DCur_A/1 -> Current_Magnitude_Squared/1(VfMDCC_DCur_A)
  Current_Magnitude_Squared/1(VfMDCC_CurMagnitudeSq_A2) -> If/1
  VfMDCC_QCur_A/1 -> Current_Magnitude_Squared/2(VfMDCC_QCur_A)

== system YMBOX_Control_Core/MDCC/MDCC_Subsystem/ElecAngle_SinCos_Adapter ==
  VfMDCC_MotElecAngle_rad : Inport  OutMin=[0]  OutMax=[4095]
  ElecAngle_Rad_To_Pu : Product  Inputs=*/
  SinCos_Service : YMBOX_SharedMath_Lib/SinCos_Service  SystemSampleTime=-1  VariantActivationTime=update diagram  AllowFlexibleInterface=on  Latency=0  AutoFrameSizeCalculation=off
  Two_Pi_Rad : Constant  Value=single(2*pi)  OutDataTypeStr=single
  VfMDCC_EAngleCos_NULL : Outport
  VfMDCC_EAngleSin_NULL : Outport  Port=2
  wires:
  SinCos_Service/2 -> VfMDCC_EAngleSin_NULL/1
  SinCos_Service/1 -> VfMDCC_EAngleCos_NULL/1
  ElecAngle_Rad_To_Pu/1 -> SinCos_Service/1
  Two_Pi_Rad/1 -> ElecAngle_Rad_To_Pu/2
  VfMDCC_MotElecAngle_rad/1 -> ElecAngle_Rad_To_Pu/1

== system YMBOX_Control_Core/MDCC/MDCC_Subsystem/Park ==
  VfMDCC_AlphaCur_A : Inport
  VfMDCC_BetaCur_A : Inport  Port=2
  VfMDCC_EAngleCos_NULL : Inport  Port=3
  VfMDCC_EAngleSin_NULL : Inport  Port=4
  Product{,1..3} (4 alike) : Product
  Subtract2 : Sum
  Subtract3 : Sum  Inputs=+-
  VfMDCC_DCur_A : Outport
  VfMDCC_QCur_A : Outport  Port=2
  wires:
  Subtract3/1 -> VfMDCC_QCur_A/1  "VfMDCC_QCur_A"
  Product3/1 -> Subtract3/2
  Product2/1 -> Subtract3/1
  Subtract2/1 -> VfMDCC_DCur_A/1  "VfMDCC_DCur_A"
  Product1/1 -> Subtract2/2
  Product/1 -> Subtract2/1
  VfMDCC_EAngleSin_NULL/1 -> Product1/2, Product3/2
  VfMDCC_BetaCur_A/1 -> Product1/1, Product2/1
  VfMDCC_EAngleCos_NULL/1 -> Product/2, Product2/2
  VfMDCC_AlphaCur_A/1 -> Product/1, Product3/1

== system YMBOX_Control_Core/MDCC/MDCC_Subsystem/UdUqCalc ==
  VeMDCC_DrvModeCmd_enum : Inport
  VfMDCC_DCur_A : Inport  Port=2
  VfMDCC_QCur_A : Inport  Port=3
  VfMDCC_DCurCmd_A : Inport  Port=4
  VfMDCC_QCurCmd_A : Inport  Port=5
  VfMDCC_MotMechSpdFiltered_rads : Inport  Port=6
  VfMDCC_PiKpValueId_NULL : Inport  Port=7
  VfMDCC_PiKpValueIq_NULL : Inport  Port=8
  VfMDCC_TestUalphaUdId_NULL : Inport  Port=9
  VfMDCC_TestUbetaUqIq_NULL : Inport  Port=10
  VbMDCC_PiReset_flg : Inport  Port=11
  VuMDCC_FFEnable_enum : Inport  Port=12
  VfMDCC_k_effective_NULL : Inport  Port=13
  Merge : Merge  Inputs=3
  Merge1 : Merge  Inputs=3
  Switch Case : SwitchCase  CaseConditions={CeMDSM_DrvModeVoltDQ_enum,[CeMDSM_DrvModeOff_enum,CeMDSM_DrvModeVoltAB_enum]}
  UdUqCalc : Subsystem  TreatAsAtomicUnit=on  RTWFcnName=vPwm_MDCC_UdUqCalc1  RTWFileName=MDCC
      settings: RTWFcnNameOpts=User specified  RTWFileNameOpts=User specified  RTWMemSecFuncExecute=icache
  UdUqCalc2 : Subsystem  TreatAsAtomicUnit=on  RTWFcnName=vPwm_MDCC_UdUqCalc2  RTWFileName=MDCC
      settings: RTWFcnNameOpts=User specified  RTWFileNameOpts=User specified  RTWMemSecFuncExecute=icache
  UdUqCalc3 : Subsystem  TreatAsAtomicUnit=on  RTWFcnName=vPwm_MDCC_UdUqCalc2  RTWFileName=MDCC
      settings: RTWFcnNameOpts=User specified  RTWFileNameOpts=User specified  RTWMemSecFuncExecute=icache
  VfMDCC_VoltD_V : Outport
  VfMDCC_VoltQ_V : Outport  Port=2
  wires:
  VfMDCC_k_effective_NULL/1 -> UdUqCalc/10(VfMDCC_k_effective_NULL)  "VfMDCC_k_effective_NULL"
  VuMDCC_FFEnable_enum/1 -> UdUqCalc/9(VuMDCC_FFEnable_enum)
  VbMDCC_PiReset_flg/1 -> UdUqCalc/8(VbMDCC_PiReset_flg)
  UdUqCalc/2(VfMDCC_VoltQ_V) -> Merge1/3  "VfMDCC_VoltQ_V"
  UdUqCalc3/2(VfMDCC_VoltQ_V) -> Merge1/2  "VfMDCC_VoltQ_V"
  UdUqCalc2/2(VfMDCC_VoltQ_V) -> Merge1/1  "VfMDCC_VoltQ_V"
  UdUqCalc/1(VfMDCC_VoltD_V) -> Merge/3  "VfMDCC_VoltD_V"
  UdUqCalc3/1(VfMDCC_VoltD_V) -> Merge/2  "VfMDCC_VoltD_V"
  UdUqCalc2/1(VfMDCC_VoltD_V) -> Merge/1  "VfMDCC_VoltD_V"
  Switch Case/2 -> UdUqCalc3/Action
  Switch Case/3 -> UdUqCalc/Action
  Switch Case/1 -> UdUqCalc2/Action
  VfMDCC_TestUbetaUqIq_NULL/1 -> UdUqCalc2/2(VfMDCC_TestUbetaUqIq_NULL)
  VfMDCC_TestUalphaUdId_NULL/1 -> UdUqCalc2/1(VfMDCC_TestUalphaUdId_NULL)
  VfMDCC_QCurCmd_A/1 -> UdUqCalc/4(VfMDCC_QCurCmd_A)
  VfMDCC_QCur_A/1 -> UdUqCalc/5(VfMDCC_QCur_A)
  VfMDCC_PiKpValueIq_NULL/1 -> UdUqCalc/6(VfMDCC_PiKpValueIq_NULL)
  VfMDCC_MotMechSpdFiltered_rads/1 -> UdUqCalc/7(VfMDCC_MotMechSpdFiltered_rads)
  VfMDCC_PiKpValueId_NULL/1 -> UdUqCalc/3(VfMDCC_PiKpValueId_NULL)
  VfMDCC_DCurCmd_A/1 -> UdUqCalc/1(VfMDCC_DCurCmd_A)
  VfMDCC_DCur_A/1 -> UdUqCalc/2(VfMDCC_DCur_A)
  Merge1/1 -> VfMDCC_VoltQ_V/1  "VfMDCC_VoltQ_V"
  Merge/1 -> VfMDCC_VoltD_V/1  "VfMDCC_VoltD_V"
  VeMDCC_DrvModeCmd_enum/1 -> Switch Case/1

== system YMBOX_Control_Core/MDSA/Inverter_Nonlinearity_Voltage_Manager/Compensation_Enable_Logic ==
  modeCmd : Inport
  activeEnable : Inport  Port=2
  voltageOperationalValid : Inport  Port=3  OutDataTypeStr=boolean
  CompGate : Logic  Inputs=4  IconShape=distinctive
  ModeNonzero : RelationalOperator  Operator=~=
  RunDelay : UnitDelay  InitialCondition=false  SampleTime=-1
  TrueB : Constant  Value=true
  ZeroU16 : Constant  Value=uint16(0)
  compEnable : Outport
  runEnable : Outport  Port=2
  wires:
  CompGate/1 -> compEnable/1
  ModeNonzero/1 -> CompGate/2
  RunDelay/1 -> runEnable/1, CompGate/4
  ZeroU16/1 -> ModeNonzero/2
  TrueB/1 -> RunDelay/1
  modeCmd/1 -> ModeNonzero/1
  activeEnable/1 -> CompGate/1
  voltageOperationalValid/1 -> CompGate/3

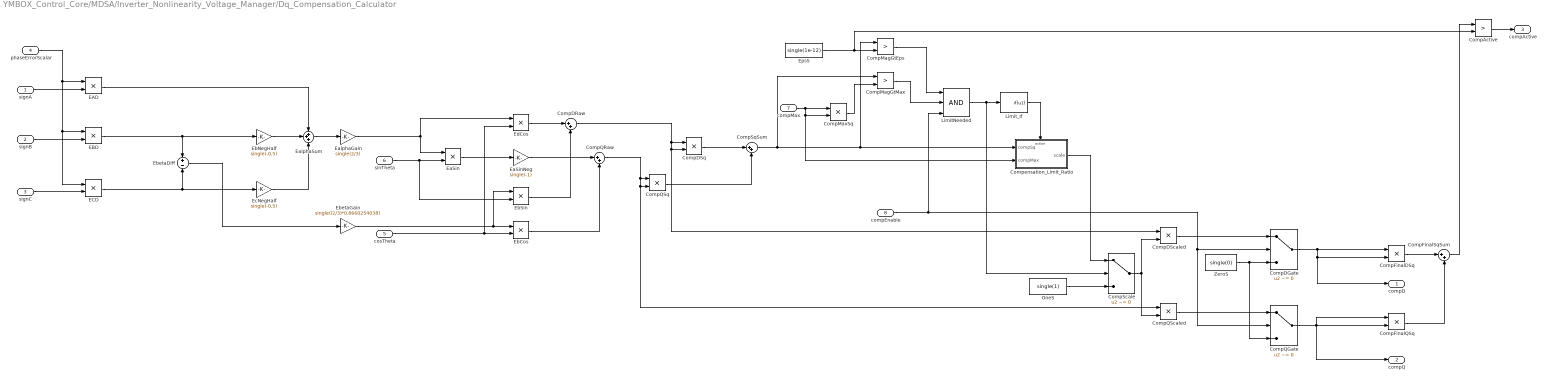
== system YMBOX_Control_Core/MDSA/Inverter_Nonlinearity_Voltage_Manager/Dq_Compensation_Calculator ==
  signA : Inport  OutDataTypeStr=single
  signB : Inport  Port=2  OutDataTypeStr=single
  signC : Inport  Port=3  OutDataTypeStr=single
  phaseErrorScalar : Inport  Port=4  OutDataTypeStr=single
  cosTheta : Inport  Port=5  OutDataTypeStr=single
  sinTheta : Inport  Port=6  OutDataTypeStr=single
  compMax : Inport  Port=7  OutDataTypeStr=single
  compEnable : Inport  Port=8  OutDataTypeStr=boolean
  CompActive : RelationalOperator  Operator=>
  CompDGate : Switch  Criteria=u2 ~= 0
  CompDRaw : Sum  Inputs=|++
  CompDScaled : Product  Inputs=**
  CompDSq : Product  Inputs=**
  CompFinalDSq : Product  Inputs=**
  CompFinalQSq : Product  Inputs=**
  CompFinalSqSum : Sum  Inputs=|++
  CompMagGtEps : RelationalOperator  Operator=>
  CompMagGtMax : RelationalOperator  Operator=>
  CompMaxSq : Product  Inputs=**
  CompQGate : Switch  Criteria=u2 ~= 0
  CompQRaw : Sum  Inputs=|++
  CompQScaled : Product  Inputs=**
  CompQSq : Product  Inputs=**
  CompScale : Switch  Criteria=u2 ~= 0
  CompSqSum : Sum  Inputs=|++
  Compensation_Limit_Ratio : Subsystem  TreatAsAtomicUnit=on
  EAD : Product  Inputs=**
  EBD : Product  Inputs=**
  ECD : Product  Inputs=**
  EaSin : Product  Inputs=**
  EaSinNeg : Gain  Gain=single(-1)
  EalphaGain : Gain  Gain=single(2/3)
  EalphaSum : Sum  Inputs=+++
  EbCos : Product  Inputs=**
  EbNegHalf : Gain  Gain=single(-0.5)
  EbSin : Product  Inputs=**
  EbetaDiff : Sum  Inputs=+-
  EbetaGain : Gain  Gain=single((2/3)*0.8660254038)
  EcNegHalf : Gain  Gain=single(-0.5)
  EdCos : Product  Inputs=**
  EpsS : Constant  Value=single(1e-12)
  LimitNeeded : Logic  Inputs=3  IconShape=distinctive
  Limit_If : If  IfExpression=u1  ShowElse=off  ZeroCross=off
  OneS : Constant  Value=single(1)
  ZeroS : Constant  Value=single(0)
  compD : Outport
  compQ : Outport  Port=2
  compActive : Outport  Port=3
  wires:
  CompActive/1 -> compActive/1
  CompFinalQSq/1 -> CompFinalSqSum/2
  CompFinalDSq/1 -> CompFinalSqSum/1
  CompQGate/1 -> CompFinalQSq/1, compQ/1, CompFinalQSq/2
  CompDGate/1 -> compD/1, CompFinalDSq/2, CompFinalDSq/1
  CompQScaled/1 -> CompQGate/1
  CompDScaled/1 -> CompDGate/1
  CompScale/1 -> CompQScaled/2, CompDScaled/2
  LimitNeeded/1 -> Limit_If/1, CompScale/2
  CompMagGtMax/1 -> LimitNeeded/2
  CompMagGtEps/1 -> LimitNeeded/1
  CompQSq/1 -> CompSqSum/2
  CompDSq/1 -> CompSqSum/1
  CompQRaw/1 -> CompQSq/1, CompQSq/2, CompQScaled/1
  EbCos/1 -> CompQRaw/2
  EaSinNeg/1 -> CompQRaw/1
  EaSin/1 -> EaSinNeg/1
  CompDRaw/1 -> CompDScaled/1, CompDSq/2, CompDSq/1
  EbSin/1 -> CompDRaw/2
  EdCos/1 -> CompDRaw/1
  EbetaDiff/1 -> EbetaGain/1
  EalphaSum/1 -> EalphaGain/1
  EcNegHalf/1 -> EalphaSum/3
  EbNegHalf/1 -> EalphaSum/2
  phaseErrorScalar/1 -> EBD/1, ECD/1, EAD/1
  compEnable/1 -> CompQGate/2, CompDGate/2, LimitNeeded/3
  signC/1 -> ECD/2
  signB/1 -> EBD/2
  signA/1 -> EAD/2
  sinTheta/1 -> EaSin/2, EbSin/2
  cosTheta/1 -> EdCos/2, EbCos/2
  EpsS/1 -> CompMagGtEps/2, CompActive/2
  OneS/1 -> CompScale/3
  ZeroS/1 -> CompQGate/3, CompDGate/3
  compMax/1 -> Compensation_Limit_Ratio/2(compMax), CompMaxSq/2, CompMaxSq/1
  CompSqSum/1 -> CompMagGtEps/1, Compensation_Limit_Ratio/1(compSq), CompMagGtMax/1
  CompMaxSq/1 -> CompMagGtMax/2
  Limit_If/1 -> Compensation_Limit_Ratio/Action
  Compensation_Limit_Ratio/1(scale) -> CompScale/1
  CompFinalSqSum/1 -> CompActive/1
  EAD/1 -> EalphaSum/1
  EBD/1 -> EbetaDiff/1, EbNegHalf/1
  ECD/1 -> EcNegHalf/1, EbetaDiff/2
  EalphaGain/1 -> EdCos/1, EaSin/1
  EbetaGain/1 -> EbSin/1, EbCos/1

== system YMBOX_Control_Core/MDSA/Inverter_Nonlinearity_Voltage_Manager/Inverter_Phase_Error_Model ==
  vdc : Inport  OutDataTypeStr=single
  deadTimeDuty : Inport  Port=2  OutDataTypeStr=single
  highDrop : Inport  Port=3  OutDataTypeStr=single
  lowDrop : Inport  Port=4  OutDataTypeStr=single
  compGain : Inport  Port=5  OutDataTypeStr=single
  polarity : Inport  Port=6  OutDataTypeStr=single
  CompScalarD : Product  Inputs=***
  DeadTerm : Product  Inputs=**
  DropSum : Sum  Inputs=|++
  HalfDrop : Gain  Gain=single(0.5)
  HighNonneg : Switch  Criteria=u2 ~= 0
  HighPos : RelationalOperator  Operator=>
  LowNonneg : Switch  Criteria=u2 ~= 0
  LowPos : RelationalOperator  Operator=>
  PhaseErrorD : Sum  Inputs=|++
  VdcNonneg : Switch  Criteria=u2 ~= 0
  VdcPos : RelationalOperator  Operator=>
  ZeroS : Constant  Value=single(0)
  phaseErrorScalar : Outport
  wires:
  CompScalarD/1 -> phaseErrorScalar/1
  HalfDrop/1 -> PhaseErrorD/2
  DropSum/1 -> HalfDrop/1
  DeadTerm/1 -> PhaseErrorD/1
  LowPos/1 -> LowNonneg/2
  HighPos/1 -> HighNonneg/2
  VdcPos/1 -> VdcNonneg/2
  ZeroS/1 -> LowPos/2, HighPos/2, LowNonneg/3, HighNonneg/3, VdcNonneg/3, VdcPos/2
  lowDrop/1 -> LowPos/1, LowNonneg/1
  highDrop/1 -> HighPos/1, HighNonneg/1
  vdc/1 -> VdcPos/1, VdcNonneg/1
  VdcNonneg/1 -> DeadTerm/1
  deadTimeDuty/1 -> DeadTerm/2
  HighNonneg/1 -> DropSum/1
  LowNonneg/1 -> DropSum/2
  PhaseErrorD/1 -> CompScalarD/1
  compGain/1 -> CompScalarD/2
  polarity/1 -> CompScalarD/3

== system YMBOX_Control_Core/MDSA/Inverter_Nonlinearity_Voltage_Manager/Managed_AlphaBeta_Calculator ==
  vdManaged : Inport
  vqManaged : Inport  Port=2
  cosTheta : Inport  Port=3
  sinTheta : Inport  Port=4
  VAlpha : Sum  Inputs=+-
  VBeta : Sum  Inputs=|++
  VdCos : Product  Inputs=**
  VdSin : Product  Inputs=**
  VqCos : Product  Inputs=**
  VqSin : Product  Inputs=**
  vAlphaManaged : Outport
  vBetaManaged : Outport  Port=2
  wires:
  VBeta/1 -> vBetaManaged/1
  VAlpha/1 -> vAlphaManaged/1
  VqCos/1 -> VBeta/2
  VdSin/1 -> VBeta/1
  VqSin/1 -> VAlpha/2
  VdCos/1 -> VAlpha/1
  vqManaged/1 -> VqSin/1, VqCos/1
  vdManaged/1 -> VdCos/1, VdSin/1
  sinTheta/1 -> VqSin/2, VdSin/2
  cosTheta/1 -> VdCos/2, VqCos/2

== system YMBOX_Control_Core/MDSA/Inverter_Nonlinearity_Voltage_Manager/Phase_Current_Sign_Manager ==
  phaseA : Inport
  phaseB : Inport  Port=2
  phaseC : Inport  Port=3
  currentBoundary : Inport  Port=4
  signHoldCount : Inport  Port=5
  runEnable : Inport  Port=6
  NegBoundary : Gain  Gain=single(-1)
  Phase_A_Sign_Hold : Subsystem
  Phase_B_Sign_Hold : Subsystem
  Phase_C_Sign_Hold : Subsystem
  signA : Outport
  signB : Outport  Port=2
  signC : Outport  Port=3
  wires:
  Phase_C_Sign_Hold/1(phaseSign) -> signC/1
  phaseC/1 -> Phase_C_Sign_Hold/1(phaseCurrent)
  Phase_B_Sign_Hold/1(phaseSign) -> signB/1
  phaseB/1 -> Phase_B_Sign_Hold/1(phaseCurrent)
  Phase_A_Sign_Hold/1(phaseSign) -> signA/1
  runEnable/1 -> Phase_A_Sign_Hold/5(runEnable), Phase_C_Sign_Hold/5(runEnable), Phase_B_Sign_Hold/5(runEnable)
  signHoldCount/1 -> Phase_A_Sign_Hold/4(signHoldCount), Phase_C_Sign_Hold/4(signHoldCount), Phase_B_Sign_Hold/4(signHoldCount)
  NegBoundary/1 -> Phase_C_Sign_Hold/3(negBoundary), Phase_A_Sign_Hold/3(negBoundary), Phase_B_Sign_Hold/3(negBoundary)
  phaseA/1 -> Phase_A_Sign_Hold/1(phaseCurrent)
  currentBoundary/1 -> NegBoundary/1, Phase_B_Sign_Hold/2(posBoundary), Phase_C_Sign_Hold/2(posBoundary), Phase_A_Sign_Hold/2(posBoundary)

== system YMBOX_Control_Core/MDSA/Inverter_Nonlinearity_Voltage_Manager/Voltage_Vector_Limiter ==
  vdRaw : Inport  OutDataTypeStr=single
  vqRaw : Inport  Port=2  OutDataTypeStr=single
  compD : Inport  Port=3  OutDataTypeStr=single
  compQ : Inport  Port=4  OutDataTypeStr=single
  vdqMaxPerVdc : Inport  Port=5  OutDataTypeStr=single
  limitEnable : Inport  Port=6  OutDataTypeStr=boolean
  vdc : Inport  Port=7  OutDataTypeStr=single
  runEnable : Inport  Port=8  OutDataTypeStr=boolean
  LimitEnableScale : Switch  Criteria=u2 ~= 0
  LimitScale : Switch  Criteria=u2 ~= 0
  LimitScaleRaw : Product  Inputs=*/
  OneS : Constant  Value=single(1)
  RunEnableScale : Switch  Criteria=u2 ~= 0
  UtilD : Product  Inputs=*/
  UtilRun : Switch  Criteria=u2 ~= 0
  VMagD : YMBOX_SharedMath_Lib/Sqrt_Service  SystemSampleTime=-1  VariantActivationTime=update diagram  AllowFlexibleInterface=on  Latency=0  AutoFrameSizeCalculation=off
  VMagGtVmax : RelationalOperator  Operator=>
  VMagSafe : Saturate  UpperLimit=inf  LowerLimit=single(1e-6)
  VPreSqSum : Sum  Inputs=|++  OutMin=0
  VdPre : Sum  Inputs=|++
  VdPreSq : Product  Inputs=**
  VdScaled : Product  Inputs=**
  VmaxRawD : Product  Inputs=**
  VoltageLimitedLogic : Logic  Inputs=3  IconShape=distinctive
  VqPre : Sum  Inputs=|++
  VqPreSq : Product  Inputs=**
  VqScaled : Product  Inputs=**
  ZeroS : Constant  Value=single(0)
  vdManaged : Outport
  vqManaged : Outport  Port=2
  voltageUtilization : Outport  Port=3
  voltageLimited : Outport  Port=4
  kMgr : Outport  Port=5
  wires:
  vdRaw/1 -> VdPre/1
  compD/1 -> VdPre/2
  VqPreSq/1 -> VPreSqSum/2
  vqRaw/1 -> VqPre/1
  LimitEnableScale/1 -> RunEnableScale/1, kMgr/1
  VqPre/1 -> VqScaled/2, VqPreSq/2, VqPreSq/1
  compQ/1 -> VqPre/2
  VdPre/1 -> VdPreSq/2, VdPreSq/1, VdScaled/1
  VdPreSq/1 -> VPreSqSum/1
  vdc/1 -> VmaxRawD/1
  VmaxRawD/1 -> VMagGtVmax/2, UtilD/2, LimitScaleRaw/1
  vdqMaxPerVdc/1 -> VmaxRawD/2
  VMagSafe/1 -> LimitScaleRaw/2
  UtilD/1 -> UtilRun/1
  VMagGtVmax/1 -> LimitScale/2, VoltageLimitedLogic/1
  LimitScaleRaw/1 -> LimitScale/1
  OneS/1 -> LimitScale/3, LimitEnableScale/3
  limitEnable/1 -> LimitEnableScale/2, VoltageLimitedLogic/2
  VoltageLimitedLogic/1 -> voltageLimited/1
  runEnable/1 -> VoltageLimitedLogic/3, UtilRun/2, RunEnableScale/2
  LimitScale/1 -> LimitEnableScale/1
  ZeroS/1 -> RunEnableScale/3, UtilRun/3
  UtilRun/1 -> voltageUtilization/1
  RunEnableScale/1 -> VdScaled/2, VqScaled/1
  VdScaled/1 -> vdManaged/1
  VqScaled/1 -> vqManaged/1
  VPreSqSum/1 -> VMagD/1
  VMagD/1 -> VMagGtVmax/1, UtilD/1, VMagSafe/1

== system YMBOX_Control_Core/MDSA/MDSA_Subsystem/PwmOutput ==
  VeMDSA_DrvModeCmd_enum : Inport
  VfMDSA_VoltAlpha_V : Inport  Port=2
  VfMDSA_VoltBeta_V : Inport  Port=3
  VfMDSA_DCBusVolt_V : Inport  Port=4
  VbMDFM_VoltageOperationalValid_flg : Inport  Port=5  OutDataTypeStr=boolean
  Arithmetic_Zero_V : Constant  Value=single(0)  OutDataTypeStr=single
  DCBus_Positive : RelationalOperator  Operator=>
  DcBus_Squared : Product  Inputs=**
  If : If  IfExpression=u1
  Merge{,1..3} (4 alike) : Merge
  Mode_Is_Active : RelationalOperator  Operator=~=
  Mode_Zero : Constant  Value=uint16(0)  OutDataTypeStr=uint16
  PwmDisable : Subsystem  TreatAsAtomicUnit=on
      settings: RTWMemSecFuncExecute=icache
  PwmEnable : Subsystem  TreatAsAtomicUnit=on
      settings: RTWMemSecFuncExecute=icache
  Pwm_Request_Is_Valid : Logic  Inputs=4
  VoltAlpha_Squared : Product  Inputs=**
  VoltBeta_Squared : Product  Inputs=**
  Voltage_Vector_Is_Bounded : RelationalOperator  Operator=<=
  Voltage_Vector_Squared : Sum
  VfMDSA_PwmDutyCyclePhaseU_NULL : Outport
  VfMDSA_PwmDutyCyclePhaseV_NULL : Outport  Port=2
  VfMDSA_PwmDutyCyclePhaseW_NULL : Outport  Port=3
  VfMDSA_k_svm_NULL : Outport  Port=4
  wires:
  PwmEnable/4(VfMDSA_k_svm_NULL) -> Merge3/2
  PwmDisable/4(VfMDSA_k_svm_NULL) -> Merge3/1
  PwmDisable/3(VfMDSA_PwmDutyCyclePhaseW_NULL) -> Merge2/1
  PwmEnable/3(VfMDSA_PwmDutyCyclePhaseW_NULL) -> Merge2/2
  PwmEnable/2(VfMDSA_PwmDutyCyclePhaseV_NULL) -> Merge1/2
  PwmDisable/2(VfMDSA_PwmDutyCyclePhaseV_NULL) -> Merge1/1
  PwmEnable/1(VfMDSA_PwmDutyCyclePhaseU_NULL) -> Merge/2
  PwmDisable/1(VfMDSA_PwmDutyCyclePhaseU_NULL) -> Merge/1
  Merge3/1 -> VfMDSA_k_svm_NULL/1
  Merge2/1 -> VfMDSA_PwmDutyCyclePhaseW_NULL/1
  Merge1/1 -> VfMDSA_PwmDutyCyclePhaseV_NULL/1
  Merge/1 -> VfMDSA_PwmDutyCyclePhaseU_NULL/1
  If/1 -> PwmEnable/Action
  VfMDSA_DCBusVolt_V/1 -> DCBus_Positive/1, PwmEnable/3(VfMDSA_DCBusVolt_V), DcBus_Squared/2, DcBus_Squared/1
  VfMDSA_VoltBeta_V/1 -> VoltBeta_Squared/1, VoltBeta_Squared/2, PwmEnable/2(VfMDSA_VoltBeta_V)
  VfMDSA_VoltAlpha_V/1 -> VoltAlpha_Squared/2, VoltAlpha_Squared/1, PwmEnable/1(VfMDSA_VoltAlpha_V)
  VeMDSA_DrvModeCmd_enum/1 -> Mode_Is_Active/1
  Mode_Zero/1 -> Mode_Is_Active/2
  Arithmetic_Zero_V/1 -> DCBus_Positive/2
  Mode_Is_Active/1 -> Pwm_Request_Is_Valid/1
  Pwm_Request_Is_Valid/1 -> If/1
  If/2 -> PwmDisable/Action
  VoltAlpha_Squared/1 -> Voltage_Vector_Squared/1
  VoltBeta_Squared/1 -> Voltage_Vector_Squared/2
  Voltage_Vector_Squared/1 -> Voltage_Vector_Is_Bounded/1
  DcBus_Squared/1 -> Voltage_Vector_Is_Bounded/2
  Voltage_Vector_Is_Bounded/1 -> Pwm_Request_Is_Valid/4
  VbMDFM_VoltageOperationalValid_flg/1 -> Pwm_Request_Is_Valid/2
  DCBus_Positive/1 -> Pwm_Request_Is_Valid/3

== system YMBOX_Control_Core/MDSA/MDSA_Subsystem/UalphaUbetaCalc ==
  VeMDSA_DrvModeCmd_enum : Inport
  VfMDSA_VoltD_V : Inport  Port=2
  VfMDSA_VoltQ_V : Inport  Port=3
  VfMDSA_MotElecAngle_rad : Inport  Port=4
  VfMDSA_MotElecSpd_rads : Inport  Port=5
  VfMDSA_PwmFreq_Hz : Inport  Port=6
  VfMDSA_TestUalphaUdId_NULL : Inport  Port=7
  VfMDSA_TestUbetaUqIq_NULL : Inport  Port=8
  If : If  IfExpression=u1 == 0
  Merge : Merge
  Merge1 : Merge
  Subsystem : Subsystem
  UalphaUbetaCalc2 : Subsystem  TreatAsAtomicUnit=on
  VfMDSA_VoltAlpha_V : Outport
  VfMDSA_VoltBeta_V : Outport  Port=2
  wires:
  If/1 -> UalphaUbetaCalc2/Action
  If/2 -> Subsystem/Action
  VfMDSA_TestUbetaUqIq_NULL/1 -> Subsystem/8(VfMDSA_TestUbetaUqIq_NULL)
  Subsystem/2(VfMDSA_VoltBeta_V) -> Merge1/2
  Merge1/1 -> VfMDSA_VoltBeta_V/1  "VfMDSA_VoltBeta_V"
  UalphaUbetaCalc2/2(VfMDSA_VoltBeta_V) -> Merge1/1
  Subsystem/1(VfMDSA_VoltAlpha_V) -> Merge/2
  Merge/1 -> VfMDSA_VoltAlpha_V/1  "VfMDSA_VoltAlpha_V"
  UalphaUbetaCalc2/1(VfMDSA_VoltAlpha_V) -> Merge/1
  VfMDSA_TestUalphaUdId_NULL/1 -> Subsystem/7(VfMDSA_TestUalphaUdId_NULL)
  VfMDSA_PwmFreq_Hz/1 -> Subsystem/6(VfMDSA_PwmFreq_Hz)
  VfMDSA_MotElecSpd_rads/1 -> Subsystem/5(VfMDSA_MotElecSpd_rads)
  VfMDSA_MotElecAngle_rad/1 -> Subsystem/4(VfMDSA_MotElecAngle_rad)
  VfMDSA_VoltQ_V/1 -> Subsystem/3(VfMDSA_VoltQ_V)  "VfMDSA_VoltQ_V"
  VfMDSA_VoltD_V/1 -> Subsystem/2(VfMDSA_VoltD_V)  "VfMDSA_VoltD_V"
  VeMDSA_DrvModeCmd_enum/1 -> If/1, Subsystem/1(VeMDSA_DrvModeCmd_enum)
